simulink model "something_dumber"  (R2026b)
settings: Solver=ode23t  StopTime=simulation.timeSim  MaxStep=1/(5*solarPlant.converterSwitchingFrequency)  AbsTol=1e-3
PreLoadFcn:
  | run('something_dumb.mlx');
values from neighbouring files (symbols this model uses):
  P170_Imp = im(ix)    [P170_PV_Initialize.m]
  P170_Vmp = vm(ix)    [P170_PV_Initialize.m]
undefined symbols (not defined in the file or in its folder): battery, bms, bmsController, connectedLoad, dcVoltage, lunarCase, maxSoC, maxVdc, minIrrad, minSoC, minVdc, olTime, P170_T, sensor, solarPlant
libraries: nesl_utility x12, fl_lib x11, simulink x7, ee_lib x3, batteryecm_lib x1, simulink_extras x1, eePwmGenerator x1
(part 1 of 2)
settings Model: Creator=The MathWorks, Inc.  LastModifiedBy=aj26g
settings SolverCC: AutoScaleAbsTol=off
settings DataIOCC: DSMLogging=off  ReturnWorkspaceOutputs=off  SaveOutput=off  SaveTime=off  SignalLoggingName=SolarPVDCWithBattery_logDB
settings OptimizationCC: ReuseModelBlockBuffer=off
settings DebuggingCC: SymbolicDimsDataTypeCodeGenerationDiagnostic=none  UnderSpecifiedDimensionMsg=warning
settings SFSimCC: CustomCodeUndefinedFunction=UseInterfaceOnly
settings RTWCC: DLArmComputeVersion=19.05
settings SimscapeCC: SimscapeLogName=simlog_SolarPVDCWithBattery  SimscapeLogSimulationStatistics=on  SimscapeLogType=all  SimscapeUseEnergyAccounting=off

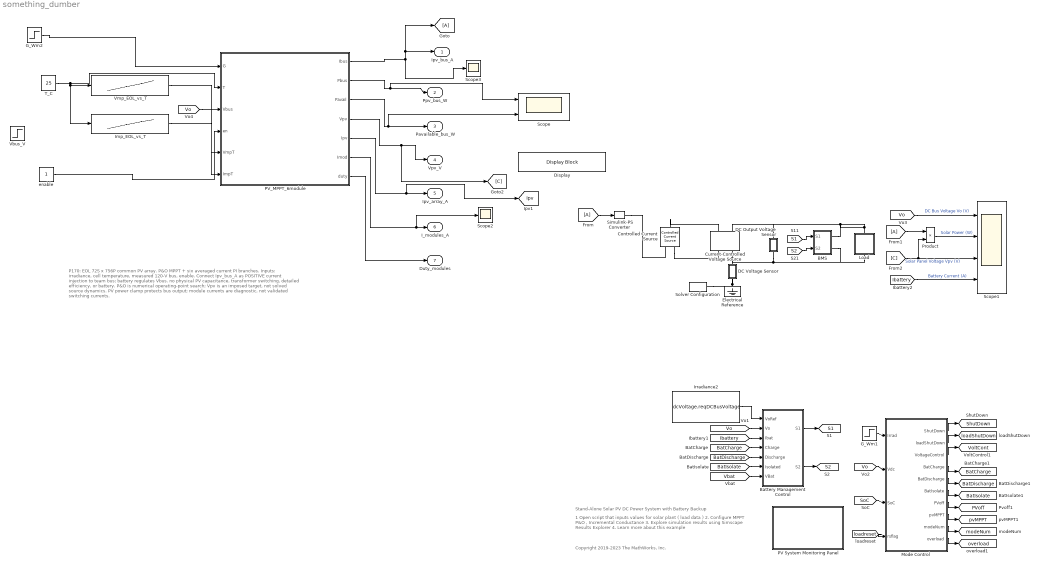
== system something_dumber ==
  note: 1 Open script that inputs values for solar plant ( load data )
      | 2. Configure MPPT P&O , Incremental Conductance
      | 3. Explore simulation results using Simscape Results Explorer
      | 4. Learn more about this example
  note: Stand-Alone Solar PV DC Power System with Battery Backup
  note: Copyright 2019-2023 The MathWorks, Inc.
  note: P170: EOL 72S x 756P common PV array. P&O MPPT + six averaged current PI branches.
      | Inputs: irradiance, cell temperature, measured 120-V bus, enable.
      | Connect Ipv_bus_A as POSITIVE current injection to team bus; battery regulates Vbus.
      |
      | no physical PV capacitance, transformer switching, detailed efficiency, or battery.
      | P&O is numerical operating-point search; Vpv is an imposed target, not solved source dynamics.
      | PV power clamp protects bus output; module currents are diagnostic, not validated switching currents.
  BMS : Subsystem
  Battery Management Control : Subsystem
  Controlled Current Source : fl_lib/Electrical/Electrical Sources/Controlled Current Source
  Current-Controlled Voltage Source : fl_lib/Electrical/Electrical Sources/Current-Controlled Voltage Source  K=1 Ohm  i1_specify=off  i1_priority=None  i1=0 A  i1_nominal_specify=off  i1_nominal_value=1  i1_nominal_unit=A  v2_specify=off  v2_priority=None  v2=0 V  v2_nominal_specify=off  v2_nominal_value=1  v2_nominal_unit=V
  DC Output Voltage Sensor : Subsystem
      mask Display: disp('v')
  DC Voltage Sensor : Subsystem
      mask Display: disp('v');
  Display : DisplayBlock  LabelPosition=Hide  Transparency=1  GridColor=[0.502, 0.502, 0.502]
  Electrical Reference : fl_lib/Electrical/Electrical Elements/Electrical Reference
  From : From
  From1 : From
  G_Wm1 : Step  Time=0.8  InitialValue=1367  FinalValue=700  SampleTime=0
  G_Wm2 : Step  Time=0.8  InitialValue=1367  FinalValue=700  SampleTime=0
  Goto : Goto
  Imp_EOL_vs_T : Lookup_n-D  NumberOfTableDimensions=1  BreakpointsForDimension1=P170_T  Table=P170_Imp  InternalRulePriority=Speed  RndMeth=Simplest
  Irradiance2 : Constant  Value=dcVoltage.reqDCBusVoltage
  Load : Subsystem
  Mode Control : Stateflow chart  TreatAsAtomicUnit=on
  PV System Monitoring Panel : Subsystem
  PV_MPPT_6module : MATLAB Function  TreatAsAtomicUnit=on
  Product : Product
  Scope : Scope  NumInputPorts=2
      settings: ActiveDisplayYMinimum=-1.4996053799360058  ActiveDisplayYMaximum=1.4239551585454688
  Scope1 : Scope  NumInputPorts=4
      settings: TimeSpan=simulation.timeSim  ActiveDisplayYMinimum=-72.27632  ActiveDisplayYMaximum=650.48692
  Scope2 : Scope
      settings: ActiveDisplayYMinimum=25.569170414602688  ActiveDisplayYMaximum=92.411823172385326  DataLoggingVariableName=ScopeData3
  Scope3 : Scope
      settings: ActiveDisplayYMinimum=153.59084488936233  ActiveDisplayYMaximum=552.88853741859577  DataLoggingVariableName=ScopeData2
  Simulink-PS Converter : nesl_utility/Simulink-PS Converter  PhysicalDomain=network_engine_domain  SubClassName=ps_input  LeftPortType=input  RightPortType=output  PseudoPeriodic=off  Frequencies=[]  NoiseDistribution=none  NoiseParameters=[]  Unit=1  AffineConversion=off  FilteringAndDerivatives=provide  SimscapeFilterOrder=1  InputFilterTimeConstant=0.001  UdotUserProvided=0
  Solver Configuration : nesl_utility/Solver Configuration  PhysicalDomain=network_engine_domain  SubClassName=solver  LeftPortType=input  RightPortType=generic  Tones=[]  Harmonics=[]  SimulateNoise=off  Profile=off  UseLocalSampling=off  EnableSwitchedLinearOptims=on  FrequencyDomain=off  UseCCode=off  RelTol=0.001  AbsTol=1e-06  MinStep=1e-09  ToWorkspace=off  RevertToSquareIcSolve=off  NumHomotopyIterations=100  PhasorMode=off  PhasorModeNumHarmonics=1  ConsistencySolver=NEWTON_FTOL  CanonicalOrdering=UNORDERED  OptimizeIntermediates=UNOPTIMIZED  MulticoreSolverChoice=BACKWARD_EULER  IndexReductionMethod=DerivativeReplacement  DoDC=off  ResidualTolerance=1e-9  ConsistencyTolSource=GLOBAL  ConsistencyAbsTol=0.001  ConsistencyRelTol=0.001  ConsistencyTolFactor=0.001  UseLocalSolver=off  LocalSolverChoice=NE_TRAPEZOIDAL_ADVANCER  ResolveIndetEquations=on  FunctionEvalNumThread=1  LocalSolverSampleTime=2e-6  DoFixedCost=off  MaxNonlinIter=10  MaxModeIter=2  ComputeImpulses=off  ImpulseIterations=2  LinearAlgebra=auto  LinearAlgebraNumThread=0  EquationFormulation=NE_TIME_EF  DelaysMemoryBudget=1024  AutomaticFiltering=on  FilteringTimeConstant=0.001  PartitionStorageMethod=AS_NEEDED  PartitionMemoryBudget=1024  PartitionMethod=FAST  MultibodyUseLocalSolver=off  MultibodyLocalSolverChoice=ODE1  MultibodyLocalSolverSampleTime=0.001
  T_C : Constant  Value=25
  Vbus_V : Step  Time=1.2  InitialValue=120  FinalValue=115  SampleTime=0
  Vmp_EOL_vs_T : Lookup_n-D  NumberOfTableDimensions=1  BreakpointsForDimension1=P170_T  Table=P170_Vmp  InternalRulePriority=Speed  RndMeth=Simplest
  enable : Constant
  Ipv_bus_A : Outport
  Ppv_bus_W : Outport  Port=2
  Pavailable_bus_W : Outport  Port=3
  Vpv_V : Outport  Port=4
  Ipv_array_A : Outport  Port=5
  I_modules_A : Outport  Port=6
  Duty_modules : Outport  Port=7
  tag scope: BatCharge=global, BatDischarge=global, BatIsolate=global, Ipv=global, PVoff=global, S1=global, S2=global, ShutDown=global, VoltCont=global, loadShutDown=global, modeNum=global, overload=global, pvMPPT=global
  wires:
  Mode Control/5(BatDischarge) -> [BatDischarge]
  [C] -> Scope1/3, Product/2  "Solar Panel Voltage Vpv (V)"
  Battery Management Control/2(S2) -> [S2]
  [Ibattery] -> Battery Management Control/3(Ibat)
  Product/1 -> Scope1/2  "Solar Power (W)"
  [Vbat] -> Battery Management Control/7(VBat)
  Mode Control/2(loadShutDown) -> [loadShutDown]
  Mode Control/9(modeNum) -> [modeNum]
  [BatDischarge] -> Battery Management Control/5(Discharge)
  Mode Control/10(overload) -> [overload]
  From1/1 -> Product/1
  Mode Control/1(ShutDown) -> [ShutDown]
  Mode Control/3(VoltageControl) -> [VoltCont]
  [BatIsolate] -> Battery Management Control/6(Isolated)
  [Vo] -> Mode Control/2(Vdc)
  Mode Control/8(pvMPPT) -> [pvMPPT]
  [loadreset] -> Mode Control/4(rsflag)
  [SoC] -> Mode Control/3(SoC)
  Mode Control/6(BatIsolate) -> [BatIsolate]
  Irradiance2/1 -> Battery Management Control/1(VoRef)
  G_Wm1/1 -> Mode Control/1(Irrad)
  Mode Control/7(PVoff) -> [PVoff]
  [Vo] -> Scope1/1  "DC Bus Voltage Vo (V)"
  Mode Control/4(BatCharge) -> [BatCharge]
  Battery Management Control/1(S1) -> [S1]
  [Ibattery] -> Scope1/4  "Battery Current (A)"
  [Vo] -> Battery Management Control/2(Vo)
  [S2] -> BMS/2(S2)
  [BatCharge] -> Battery Management Control/4(Charge)
  [S1] -> BMS/1(S1)
  PV_MPPT_6module/6(Imod) -> Scope2/1, I_modules_A/1
  PV_MPPT_6module/1(Ibus) -> Scope3/1, Goto/1, Ipv_bus_A/1
  G_Wm2/1 -> PV_MPPT_6module/1(G)
  PV_MPPT_6module/4(Vpv) -> [C], Vpv_V/1
  PV_MPPT_6module/5(Ipv) -> [Ipv], Ipv_array_A/1
  PV_MPPT_6module/7(duty) -> Duty_modules/1
  Imp_EOL_vs_T/1 -> PV_MPPT_6module/6(ImpT)
  PV_MPPT_6module/3(Pavail) -> Scope/2, Pavailable_bus_W/1
  enable/1 -> PV_MPPT_6module/4(en)
  PV_MPPT_6module/2(Pbus) -> Scope/1, Ppv_bus_W/1
  T_C/1 -> Vmp_EOL_vs_T/1, Imp_EOL_vs_T/1, PV_MPPT_6module/2(T)
  Vmp_EOL_vs_T/1 -> PV_MPPT_6module/5(VmpT)
  From/1 -> Simulink-PS Converter/1
  [Vo] -> PV_MPPT_6module/3(Vbus)
  connections:
  Load/LConn1 -- DC Output Voltage Sensor/RConn1 -- Current-Controlled Voltage Source/LConn2 -- BMS/RConn1
  Solver Configuration/RConn1 -- Electrical Reference/LConn1 -- DC Voltage Sensor/LConn1
  BMS/RConn2 -- Load/RConn1 -- Current-Controlled Voltage Source/RConn2 -- DC Voltage Sensor/RConn1 -- DC Output Voltage Sensor/LConn1
  Simulink-PS Converter/RConn1 -- Controlled Current Source/RConn1
  Controlled Current Source/LConn1 -- Current-Controlled Voltage Source/LConn1
  Controlled Current Source/RConn2 -- Current-Controlled Voltage Source/RConn1

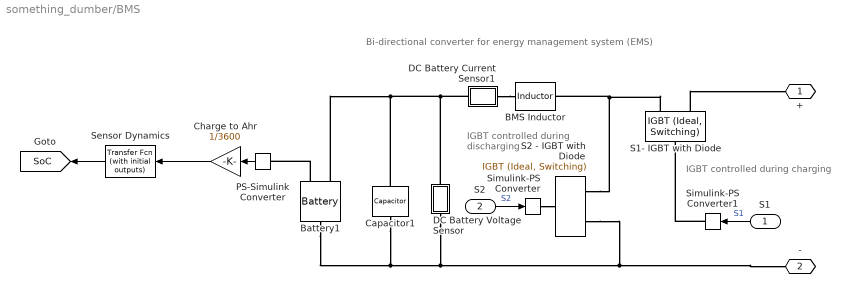
== system something_dumber/BMS ==
  note: IGBT controlled during charging
  note: Bi-directional converter for energy management system (EMS)
  note: IGBT controlled during discharging
  S1 : Inport
  S2 : Inport  Port=2
  BMS Inductor : fl_lib/Electrical/Electrical Elements/Inductor  l=bms.batteryChargingInductor H  r=bms.batteryChargingInductorResistance Ohm  g=1e-9 1/Ohm  i_specify=off  i_priority=High  i=0 A  i_nominal_specify=off  i_nominal_value=1  i_nominal_unit=A  v_specify=off  v_priority=High  v=0 V  v_nominal_specify=off  v_nominal_value=1  v_nominal_unit=V  i_L_specify=on  i_L_priority=High  i_L=0 A  i_L_nominal_specify=off  i_L_nominal_value=1  i_L_nominal_unit=A
      settings: LogSimulationData=on
  Battery1 : batteryecm_lib/Battery  Vnom=battery.nominalBatteryVoltage V  prm_dir=1  R1_dis=2 Ohm  R1_ch=2 Ohm  R1=0.01 Ohm  prm_AH=2  AH=connectedLoad.batteryAmpHr hr*A  V1=battery.minBatteryNominalVoltage V  AH1=connectedLoad.batteryAmpHr*0.2 hr*A  prm_R2=2  R2=2000 Ohm  Tmeas=298.15 K  charge_measurement_port=simscape.enum.battery.enable.yes  prm_dyn=1  Rp1=0.005 Ohm  tau1=30 s  Rp2=0.005 Ohm  tau2=30 s  Rp3=0.005 Ohm  tau3=30 s  Rp4=0.005 Ohm  tau4=30 s  Rp5=0.005 Ohm  tau5=30 s  prm_fade=1  N_fade=100  AH_fade=45 hr*A  R1_fade=2.02 Ohm  R1_ch_fade=2.02 Ohm  V1_fade=10.35 V  prm_age=1  prm_age_OCV=1  OCV_age=0.9  SOC_age=60  Tmeas_age=298.15 K  delta_time_age_vec=[0] d  temperature_age_vec=[273] K  OCV_scaling_age=2.2134e6  OCV_offset_age=1.632e6  temp_exp_age=0.515833569 V  t_exp_age=0.75  Vnom_T2=12 V  R1_T2=2.2 Ohm  R1_T2_dis=2.2 Ohm  R1_T2_ch=2.2 Ohm  V1_T2=11.4 V  R2_T2=2200 Ohm  Rp1_T2=0.005 Ohm  tau1_T2=30 s  Rp2_T2=0.005 Ohm  tau2_T2=30 s  Rp3_T2=0.005 Ohm  tau3_T2=30 s  Rp4_T2=0.005 Ohm  tau4_T2=30 s  Rp5_T2=0.005 Ohm  tau5_T2=30 s  Tmeas2=273.15 K  thermal_port=simscape.enum.thermaleffects.omit  thermal_mass=30000 J/K  i_specify=off  i_priority=None  i=0 A  i_nominal_specify=off  i_nominal_value=1  i_nominal_unit=A  v_specify=off  v_priority=None  v=0 V  v_nominal_specify=off  v_nominal_value=1  v_nominal_unit=V  charge_specify=on  charge_priority=High  charge=batteryInitialStateOfCharge hr*A  charge_nominal_specify=off  charge_nominal_value=1  charge_nominal_unit=A*hr  num_cycles_specify=off  num_cycles_priority=High  num_cycles=0  num_cycles_nominal_specify=off  num_cycles_nominal_value=1  num_cycles_nominal_unit=1  temperature_specify=off  temperature_priority=High  temperature=298.15 K  temperature_nominal_specify=off  temperature_nominal_value=1  temperature_nominal_unit=K
  Capacitor1 : fl_lib/Electrical/Electrical Elements/Capacitor  c=boost.outputCapacitor F  r=1e-6 Ohm  g=0 1/Ohm  i_specify=off  i_priority=None  i=0 A  i_nominal_specify=off  i_nominal_value=1  i_nominal_unit=A  v_specify=off  v_priority=None  v=0 V  v_nominal_specify=off  v_nominal_value=1  v_nominal_unit=V  vc_specify=on  vc_priority=High  vc=batteryInputCapacitorInitialVoltage V  vc_nominal_specify=off  vc_nominal_value=1  vc_nominal_unit=V
  Charge to Ahr : Gain  Gain=1/3600
  DC Battery Current Sensor1 : Subsystem
      mask Display: disp('i');
  DC Battery Voltage Sensor : Subsystem
      mask Display: disp('v');
  PS-Simulink Converter : nesl_utility/PS-Simulink Converter  PhysicalDomain=network_engine_domain  SubClassName=ps_output  LeftPortType=input  RightPortType=output  PseudoPeriodic=off  Frequencies=[]  VectorFormat=1-D array  Unit=inherit  AffineConversion=off
  S1- IGBT with Diode : ee_lib/Semiconductors & Converters/IGBT (Ideal, Switching)  port_option=ee.enum.controlport.ps  Vf=0.1 V  Ron=0.001 Ohm  Goff=1e-5 1/Ohm  Vth=2.5 V  diode_param=2  diode_Vf=0.1 V  diode_Ron=0.001 Ohm  diode_Goff=1e-5 1/Ohm  diode_C=50e-9 F  diode_iRM=-235 A  diode_iF=300 A  diode_idot=-50 A/us  diode_trr_param=1  diode_trr_factor=3  diode_trr=15 us  diode_Qrr=1500 s*uA  ice_specify=off  ice_priority=None  ice=0 A  ice_nominal_specify=off  ice_nominal_value=1  ice_nominal_unit=A  vce_specify=off  vce_priority=None  vce=0 V  vce_nominal_specify=off  vce_nominal_value=1  vce_nominal_unit=V  vge_specify=off  vge_priority=None  vge=0 V  vge_nominal_specify=off  vge_nominal_value=1  vge_nominal_unit=V  thermal_loss_option=ee.enum.converters.thermalLossOption.constantvalues  Von_data=[0, .1, .6, .8, 1, 1.3, 1.6, 2, 2.4; 0, .1, .7, 1, 1.2, 1.5, 1.9, 2.4, 2.8] V  Tj=[298.15, 398.15] K  Iout_data=[0, .1, 1, 5, 10, 20, 40, 70, 100] A  tabulateWithVce=false  Eon_data=[0, .0024, .024, .12, .2, .48, 1.04, 2.16, 3.24; 0, .003, .03, .15, .25, .6, 1.3, 2.7, 4.05] * 1e-3 J  Eoff_data=[0, .0007, .0066, .033, .066, .17, .33, .83, 1.5; 0, .001, .01, .05, .1, .25, .5, 1.2, 2.2] * 1e-3 J  Eon_data_3D=[zeros(2, 9, 3)] J  Eoff_data_3D=[zeros(2, 9, 3)] J  Tj_loss=[298.15, 398.15] K  Iout_data_loss=[0, .1, 1, 5, 10, 20, 40, 70, 100] A  Vce_loss=[0, 150, 300] V  Eon_scalar=22.86e-3 J  Eoff_scalar=17.14e-3 J  Voff=300 V  Iout_scalar=600 A  useCurrentFromPreviousCycle=true  currentMeasDelay=0 s  useVoltageFromPreviousCycle=true  voltageMeasDelay=0 s  diodeModelType=ee.enum.converters.diodeModelType.pwl  diodeTableType=ee.enum.diode.tableType.IfMat  diode_ReverseIVType=ee.enum.diode.diodeReverseIV.constant  diode_IfMat=[.07, .12, .19, 1.75, 4.24, 7.32, 11.2; .16, .3, .72, 2.14, 4.02, 6.35, 9.12] A  diode_VfMat=[.9, 1.15, 1.25, 1.5, 1.75, 2.17, 2.6, 2.85; .58, .68, .75, 1.1, 1.38, 1.77, 2.27, 2.7] V  diode_TjVec=[25, 125] degC  diode_VfVec=[.5, .7, .9, 1.3, 1.7, 2.1, 2.5] V  diode_IfVec=[.1, .2, .5, 1, 2, 4, 7, 10] A  diode_IrMat=[1e-06, 2e-06, 5e-06, 1e-05, 2.5e-05, 5e-05, .0001; 2e-06, 5e-06, 1e-05, 4e-05, 8e-05, .0002, .0005] A  diode_VrMat=[10, 100, 200, 250, 300, 325, 350; 10, 70, 160, 220, 270, 300, 320] V  diode_VrVec=[10, 20, 40, 50, 70, 80, 100] V  diode_IrVec=[1e-06, 2e-06, 5e-06, 1e-05, 2e-05, 5e-05, .0001] A  diode_Vr=-600 V  diode_Ls=150 nH  diode_Erec=0.03 J  diode_rec_loss_model=ee.enum.diode.reverseRecoveryModelTabulateUpTo3D.fixed  diode_ErecVal=0 J  diode_scaleWithIandV=true  diode_ErecMat=zeros(2, 3) J  diodeErecMat3D=zeros(2, 3, 2) J  diode_TjrecVec=[298.15, 398.15] K  diode_IfrecVec=[.1, 1, 10] A  diodeVrecVec=[0, 100] V  diode_IrecVal=10 A  diode_VrecVal=10 V  diode_tFilter=1 / 1000 / 100 s  separateThermalPortForDiode=false  thermal_network_parameterization=ee.enum.thermalNetworkTopology.external  Rth=[.08, .5] K/W  Rth_Cauer=[.08, .1, .5] K/W  Rth_Foster=[.08, .14, .22, .16] K/W  thermal_mass_parameterization=ee.enum.thermalNetwork.timeconstant  thermal_mass=[.01, .5] J/K  thermal_mass_Cauer=[.01, .1, .5] J/K  thermal_mass_Foster=[.001, .005, .05, .5] J/K  thermal_time_constant=[.001, .2] s  thermal_time_constant_Cauer=[.001, .1, .2] s  thermal_time_constant_Foster=[7e-05, .0007, .01, .08] s  thermal_mass_initial_temperatures=[25, 25] degC  thermal_mass_initial_temperatures_Cauer=[25, 25, 25] degC  junction_thermal_mass=0.01 J/K  Tvec_initial_Foster=[25, 25, 25, 25] degC  RthDiode=[.03, .2] K/W  RthCauerDiode=[.03, .1, .2] K/W  RthFosterDiode=[.03, .2] K/W  thermalMassDiode=[3, 25] J/K  thermalMassCauerDiode=[3, 10, 25] J/K  thermalMassFosterDiode=[33, 50] J/K  thermalTauDiode=[.1, 5] s  thermalTauCauerDiode=[.1, 1, 5] s  thermalTauFosterDiode=[1, 10] s  thermalMassInitTempDiode=[25, 25] degC  thermalMassInitTempCauerDiode=[25, 25, 25] degC  junctionthermalMassDiode=0.1 J/K  TVecInitialFosterDiode=[25, 25] degC  no_thermal_network=0  IGBT_junction_temperature_specify=off  IGBT_junction_temperature_priority=None  IGBT_junction_temperature=25 degC  IGBT_junction_temperature_nominal_specify=off  IGBT_junction_temperature_nominal_value=1  IGBT_junction_temperature_nominal_unit=degC  diode_junction_temperature_specify=off  diode_junction_temperature_priority=None  diode_junction_temperature=25 degC  diode_junction_temperature_nominal_specify=off  diode_junction_temperature_nominal_value=1  diode_junction_temperature_nominal_unit=degC  Qj_specify=off  Qj_priority=None  Qj=0 W  Qj_nominal_specify=off  Qj_nominal_value=1  Qj_nominal_unit=W  accumulatedSwitchingLosses_specify=off  accumulatedSwitchingLosses_priority=None  accumulatedSwitchingLosses=0 J
  S2 - IGBT with Diode : ee_lib/Semiconductors & Converters/IGBT (Ideal, Switching)  port_option=ee.enum.controlport.ps  Vf=0.1 V  Ron=0.001 Ohm  Goff=1e-5 1/Ohm  Vth=2.5 V  diode_param=2  diode_Vf=0.1 V  diode_Ron=0.001 Ohm  diode_Goff=1e-5 1/Ohm  diode_C=50e-9 F  diode_iRM=-235 A  diode_iF=300 A  diode_idot=-50 A/us  diode_trr_param=1  diode_trr_factor=3  diode_trr=15 us  diode_Qrr=1500 s*uA  ice_specify=off  ice_priority=None  ice=0 A  ice_nominal_specify=off  ice_nominal_value=1  ice_nominal_unit=A  vce_specify=off  vce_priority=None  vce=0 V  vce_nominal_specify=off  vce_nominal_value=1  vce_nominal_unit=V  vge_specify=off  vge_priority=None  vge=0 V  vge_nominal_specify=off  vge_nominal_value=1  vge_nominal_unit=V  thermal_loss_option=ee.enum.converters.thermalLossOption.constantvalues  Von_data=[0, .1, .6, .8, 1, 1.3, 1.6, 2, 2.4; 0, .1, .7, 1, 1.2, 1.5, 1.9, 2.4, 2.8] V  Tj=[298.15, 398.15] K  Iout_data=[0, .1, 1, 5, 10, 20, 40, 70, 100] A  tabulateWithVce=false  Eon_data=[0, .0024, .024, .12, .2, .48, 1.04, 2.16, 3.24; 0, .003, .03, .15, .25, .6, 1.3, 2.7, 4.05] * 1e-3 J  Eoff_data=[0, .0007, .0066, .033, .066, .17, .33, .83, 1.5; 0, .001, .01, .05, .1, .25, .5, 1.2, 2.2] * 1e-3 J  Eon_data_3D=[zeros(2, 9, 3)] J  Eoff_data_3D=[zeros(2, 9, 3)] J  Tj_loss=[298.15, 398.15] K  Iout_data_loss=[0, .1, 1, 5, 10, 20, 40, 70, 100] A  Vce_loss=[0, 150, 300] V  Eon_scalar=22.86e-3 J  Eoff_scalar=17.14e-3 J  Voff=300 V  Iout_scalar=600 A  useCurrentFromPreviousCycle=true  currentMeasDelay=0 s  useVoltageFromPreviousCycle=true  voltageMeasDelay=0 s  diodeModelType=ee.enum.converters.diodeModelType.pwl  diodeTableType=ee.enum.diode.tableType.IfMat  diode_ReverseIVType=ee.enum.diode.diodeReverseIV.constant  diode_IfMat=[.07, .12, .19, 1.75, 4.24, 7.32, 11.2; .16, .3, .72, 2.14, 4.02, 6.35, 9.12] A  diode_VfMat=[.9, 1.15, 1.25, 1.5, 1.75, 2.17, 2.6, 2.85; .58, .68, .75, 1.1, 1.38, 1.77, 2.27, 2.7] V  diode_TjVec=[25, 125] degC  diode_VfVec=[.5, .7, .9, 1.3, 1.7, 2.1, 2.5] V  diode_IfVec=[.1, .2, .5, 1, 2, 4, 7, 10] A  diode_IrMat=[1e-06, 2e-06, 5e-06, 1e-05, 2.5e-05, 5e-05, .0001; 2e-06, 5e-06, 1e-05, 4e-05, 8e-05, .0002, .0005] A  diode_VrMat=[10, 100, 200, 250, 300, 325, 350; 10, 70, 160, 220, 270, 300, 320] V  diode_VrVec=[10, 20, 40, 50, 70, 80, 100] V  diode_IrVec=[1e-06, 2e-06, 5e-06, 1e-05, 2e-05, 5e-05, .0001] A  diode_Vr=-600 V  diode_Ls=150 nH  diode_Erec=0.03 J  diode_rec_loss_model=ee.enum.diode.reverseRecoveryModelTabulateUpTo3D.fixed  diode_ErecVal=0 J  diode_scaleWithIandV=true  diode_ErecMat=zeros(2, 3) J  diodeErecMat3D=zeros(2, 3, 2) J  diode_TjrecVec=[298.15, 398.15] K  diode_IfrecVec=[.1, 1, 10] A  diodeVrecVec=[0, 100] V  diode_IrecVal=10 A  diode_VrecVal=10 V  diode_tFilter=1 / 1000 / 100 s  separateThermalPortForDiode=false  thermal_network_parameterization=ee.enum.thermalNetworkTopology.external  Rth=[.08, .5] K/W  Rth_Cauer=[.08, .1, .5] K/W  Rth_Foster=[.08, .14, .22, .16] K/W  thermal_mass_parameterization=ee.enum.thermalNetwork.timeconstant  thermal_mass=[.01, .5] J/K  thermal_mass_Cauer=[.01, .1, .5] J/K  thermal_mass_Foster=[.001, .005, .05, .5] J/K  thermal_time_constant=[.001, .2] s  thermal_time_constant_Cauer=[.001, .1, .2] s  thermal_time_constant_Foster=[7e-05, .0007, .01, .08] s  thermal_mass_initial_temperatures=[25, 25] degC  thermal_mass_initial_temperatures_Cauer=[25, 25, 25] degC  junction_thermal_mass=0.01 J/K  Tvec_initial_Foster=[25, 25, 25, 25] degC  RthDiode=[.03, .2] K/W  RthCauerDiode=[.03, .1, .2] K/W  RthFosterDiode=[.03, .2] K/W  thermalMassDiode=[3, 25] J/K  thermalMassCauerDiode=[3, 10, 25] J/K  thermalMassFosterDiode=[33, 50] J/K  thermalTauDiode=[.1, 5] s  thermalTauCauerDiode=[.1, 1, 5] s  thermalTauFosterDiode=[1, 10] s  thermalMassInitTempDiode=[25, 25] degC  thermalMassInitTempCauerDiode=[25, 25, 25] degC  junctionthermalMassDiode=0.1 J/K  TVecInitialFosterDiode=[25, 25] degC  no_thermal_network=0  IGBT_junction_temperature_specify=off  IGBT_junction_temperature_priority=None  IGBT_junction_temperature=25 degC  IGBT_junction_temperature_nominal_specify=off  IGBT_junction_temperature_nominal_value=1  IGBT_junction_temperature_nominal_unit=degC  diode_junction_temperature_specify=off  diode_junction_temperature_priority=None  diode_junction_temperature=25 degC  diode_junction_temperature_nominal_specify=off  diode_junction_temperature_nominal_value=1  diode_junction_temperature_nominal_unit=degC  Qj_specify=off  Qj_priority=None  Qj=0 W  Qj_nominal_specify=off  Qj_nominal_value=1  Qj_nominal_unit=W  accumulatedSwitchingLosses_specify=off  accumulatedSwitchingLosses_priority=None  accumulatedSwitchingLosses=0 J
  Sensor Dynamics : simulink_extras/Additional Linear/Transfer Fcn (with initial outputs)  N=[1]  D=[1/sensor.samplingFreq 1]  Y0=minSoC  U0=0
  Simulink-PS Converter : nesl_utility/Simulink-PS Converter  PhysicalDomain=network_engine_domain  SubClassName=ps_input  LeftPortType=input  RightPortType=output  PseudoPeriodic=off  Frequencies=[]  NoiseDistribution=none  NoiseParameters=[]  Unit=1  AffineConversion=off  FilteringAndDerivatives=provide  SimscapeFilterOrder=1  InputFilterTimeConstant=0.001  UdotUserProvided=0
  Simulink-PS Converter1 : nesl_utility/Simulink-PS Converter  PhysicalDomain=network_engine_domain  SubClassName=ps_input  LeftPortType=input  RightPortType=output  PseudoPeriodic=off  Frequencies=[]  NoiseDistribution=none  NoiseParameters=[]  Unit=1  AffineConversion=off  FilteringAndDerivatives=provide  SimscapeFilterOrder=1  InputFilterTimeConstant=0.001  UdotUserProvided=0
  + : PMIOPort  Side=Right
  - : PMIOPort  Port=2  Side=Right
  tag scope: SoC=global
  wires:
  S2/1 -> Simulink-PS Converter/1  "S2"
  S1/1 -> Simulink-PS Converter1/1  "S1"
  PS-Simulink Converter/1 -> Charge to Ahr/1
  Sensor Dynamics/1 -> [SoC]
  Charge to Ahr/1 -> Sensor Dynamics/1
  connections:
  S2 - IGBT with Diode/RConn2 -- Battery1/RConn1 -- Capacitor1/RConn1 -- DC Battery Voltage Sensor/LConn1 -- -/RConn1
  S2 - IGBT with Diode/RConn1 -- S1- IGBT with Diode/RConn2 -- BMS Inductor/RConn1
  S1- IGBT with Diode/RConn1 -- +/RConn1
  Simulink-PS Converter/RConn1 -- S2 - IGBT with Diode/LConn1
  Battery1/LConn2 -- PS-Simulink Converter/LConn1
  Simulink-PS Converter1/RConn1 -- S1- IGBT with Diode/LConn1
  DC Battery Current Sensor1/RConn1 -- BMS Inductor/LConn1
  DC Battery Current Sensor1/LConn1 -- DC Battery Voltage Sensor/RConn1 -- Battery1/LConn1 -- Capacitor1/LConn1

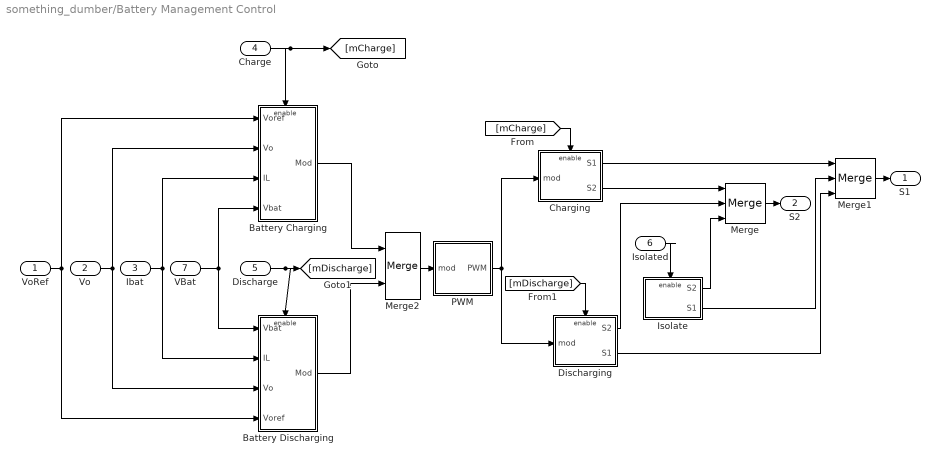
== system something_dumber/Battery Management Control ==
  VoRef : Inport
  Vo : Inport  Port=2
  Ibat : Inport  Port=3
  Charge : Inport  Port=4
  Discharge : Inport  Port=5
  Isolated : Inport  Port=6
  VBat : Inport  Port=7
  Battery Charging : Subsystem
  Battery Discharging : Subsystem
  Charging : Subsystem  TreatAsAtomicUnit=on
  Discharging : Subsystem  TreatAsAtomicUnit=on
  Isolate : Subsystem  TreatAsAtomicUnit=on
  Merge : Merge  Inputs=3
  Merge1 : Merge  Inputs=3
  Merge2 : Merge
  PWM : Subsystem
  S1 : Outport
  S2 : Outport  Port=2
  wires:
  Charging/2(S2) -> Merge/1
  Discharging/1(S2) -> Merge/2
  Charging/1(S1) -> Merge1/1
  Isolate/1(S2) -> Merge/3
  Isolate/2(S1) -> Merge1/2
  Discharging/2(S1) -> Merge1/3
  Merge1/1 -> S1/1
  Isolated/1 -> Isolate/Enable
  Vo/1 -> Battery Charging/2(Vo), Battery Discharging/3(Vo)
  Ibat/1 -> Battery Charging/3(IL), Battery Discharging/2(IL)
  Battery Charging/1(Mod) -> Merge2/1
  Battery Discharging/1(Mod) -> Merge2/2
  Merge/1 -> S2/1
  Charge/1 -> [mCharge], Battery Charging/Enable
  Discharge/1 -> Battery Discharging/Enable, [mDischarge]
  [mCharge] -> Charging/Enable
  [mDischarge] -> Discharging/Enable
  PWM/1(PWM) -> Charging/1(mod), Discharging/1(mod)
  Merge2/1 -> PWM/1(mod)
  VoRef/1 -> Battery Charging/1(Voref), Battery Discharging/4(Voref)
  VBat/1 -> Battery Discharging/1(Vbat), Battery Charging/4(Vbat)

== system something_dumber/DC Output Voltage Sensor ==
  PS-Simulink Converter : nesl_utility/PS-Simulink Converter  PhysicalDomain=network_engine_domain  SubClassName=ps_output  LeftPortType=input  RightPortType=output  PseudoPeriodic=off  Frequencies=[]  VectorFormat=1-D array  Unit=1  AffineConversion=off
  Sensor dynamics : TransferFcn  Numerator=1  Denominator=[1/sensor.samplingFreq 1]
  Voltage Sensor : fl_lib/Electrical/Electrical Sensors/Voltage Sensor
  - : PMIOPort  Side=Left
  + : PMIOPort  Port=2  Side=Right
  tag scope: Vo=global
  wires:
  PS-Simulink Converter/1 -> Sensor dynamics/1
  Sensor dynamics/1 -> [Vo]
  connections:
  Voltage Sensor/RConn2 -- -/RConn1
  Voltage Sensor/RConn1 -- PS-Simulink Converter/LConn1
  Voltage Sensor/LConn1 -- +/RConn1

== system something_dumber/DC Voltage Sensor ==
  PS-Simulink Converter : nesl_utility/PS-Simulink Converter  PhysicalDomain=network_engine_domain  SubClassName=ps_output  LeftPortType=input  RightPortType=output  PseudoPeriodic=off  Frequencies=[]  VectorFormat=1-D array  Unit=1  AffineConversion=off
  Sensor dynamics : TransferFcn  Numerator=1  Denominator=[1/sensor.samplingFreq 1]
  Voltage Sensor : fl_lib/Electrical/Electrical Sensors/Voltage Sensor
      settings: LogSimulationData=on
  - : PMIOPort  Side=Left
  + : PMIOPort  Port=2  Side=Right
  tag scope: Vpv=global
  wires:
  PS-Simulink Converter/1 -> Sensor dynamics/1
  Sensor dynamics/1 -> [Vpv]
  connections:
  Voltage Sensor/LConn1 -- +/RConn1
  Voltage Sensor/RConn1 -- PS-Simulink Converter/LConn1
  Voltage Sensor/RConn2 -- -/RConn1

== system something_dumber/Load ==
  AC Current Sensor2 : Subsystem
      mask Display: disp('i');
  Load : Subsystem
  Load Flag : Subsystem
  Load Resistance : fl_lib/Electrical/Electrical Elements/Variable Resistor  Rmin=0 Ohm  thermalEnable=false  thermal_mass=1 J/K  i_specify=off  i_priority=None  i=5 A  i_nominal_specify=off  i_nominal_value=1  i_nominal_unit=A  v_specify=off  v_priority=None  v=0 V  v_nominal_specify=off  v_nominal_value=1  v_nominal_unit=V  T_specify=off  T_priority=None  T=300 K  T_nominal_specify=off  T_nominal_value=1  T_nominal_unit=K
  SPST Switch : ee_lib/Switches & Breakers/SPST Switch  R_closed=0.01 Ohm  G_open=1e-6 S  Threshold=0.5 V  Width=0 V  model_dynamics=0  t_on=1e-3 s  t_off=1e-3 s  initial_vT=0 V
  + : PMIOPort  Side=Left
  - : PMIOPort  Port=2  Side=Right
  connections:
  +/RConn1 -- SPST Switch/LConn2
  Load Resistance/LConn2 -- AC Current Sensor2/LConn1
  Load Resistance/RConn1 -- -/RConn1
  Load/RConn1 -- Load Resistance/LConn1
  Load Flag/RConn1 -- SPST Switch/LConn1
  AC Current Sensor2/RConn1 -- SPST Switch/RConn1

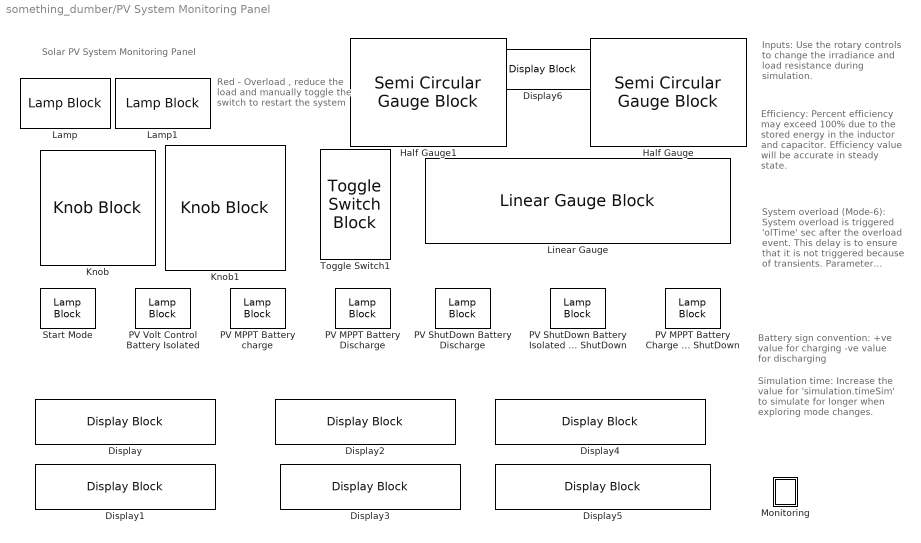
== system something_dumber/PV System Monitoring Panel ==
  note: Red - Overload , reduce the load and manually toggle the switch to restart the system
  note: Solar PV System Monitoring Panel
  note: Simulation time:
      | Increase the value for 'simulation.timeSim' to simulate for longer when exploring mode changes.
  note: Inputs:
      | Use the rotary controls to change the irradiance and load resistance during simulation.
  note: System overload (Mode-6):
      | System overload is triggered 'olTime' sec after the overload event. This delay is to ensure that it is not triggered because of transients. Parameter 'olTime' can be modified in the supporting livescript.
  note: Efficiency:
      | Percent efficiency may exceed 100% due to the stored energy in the inductor and capacitor. Efficiency value will be accurate in steady state.
  note: Battery sign convention:
      | +ve value for charging
      | -ve value for discharging
  Display{,1..6} (7 alike) : DisplayBlock  Transparency=1  GridColor=[0.502, 0.502, 0.502]
  Half Gauge : SemiCircularGaugeBlock  ScaleMin=20  FontColor=[0.0, 0.0, 0.0]
  Half Gauge1 : SemiCircularGaugeBlock  FontColor=[0.0, 0.0, 0.0]
  Knob : KnobBlock  ScaleMin=150  ScaleMax=1000
  Knob1 : KnobBlock  ScaleMin=0.15  ScaleMax=20
  Lamp : LampBlock  DefaultColor=[192.0, 192.0, 192.0]
  Lamp1 : LampBlock  DefaultColor=[192.0, 192.0, 192.0]
  Linear Gauge : LinearGaugeBlock  ScaleMin=-100  FontColor=[0.0, 0.0, 0.0]
  Monitoring : Subsystem
  PV MPPT Battery Charge Load ShutDown : LampBlock  DefaultColor=[192.0, 192.0, 192.0]
  PV MPPT Battery Discharge : LampBlock  DefaultColor=[192.0, 192.0, 192.0]
  PV MPPT Battery charge : LampBlock  DefaultColor=[192.0, 192.0, 192.0]
  PV ShutDown Battery Discharge : LampBlock  DefaultColor=[192.0, 192.0, 192.0]
  PV ShutDown Battery Isolated System ShutDown : LampBlock  DefaultColor=[192.0, 192.0, 192.0]
  PV Volt Control Battery Isolated : LampBlock  DefaultColor=[192.0, 192.0, 192.0]
  Start Mode : LampBlock  DefaultColor=[192.0, 192.0, 192.0]
  Toggle Switch1 : ToggleSwitchBlock

== system something_dumber/BMS/DC Battery Current Sensor1 ==
  Current Sensor : fl_lib/Electrical/Electrical Sensors/Current Sensor
  PS-Simulink Converter : nesl_utility/PS-Simulink Converter  PhysicalDomain=network_engine_domain  SubClassName=ps_output  LeftPortType=input  RightPortType=output  PseudoPeriodic=off  Frequencies=[]  VectorFormat=1-D array  Unit=1  AffineConversion=off
  Sensor dynamics : TransferFcn  Numerator=1  Denominator=[1/sensor.samplingFreq 1]
  - : PMIOPort  Side=Left
  + : PMIOPort  Port=2  Side=Right
  tag scope: Ibattery=global
  wires:
  PS-Simulink Converter/1 -> Sensor dynamics/1
  Sensor dynamics/1 -> [Ibattery]
  connections:
  Current Sensor/RConn1 -- PS-Simulink Converter/LConn1
  +/RConn1 -- Current Sensor/LConn1
  Current Sensor/RConn2 -- -/RConn1

== system something_dumber/BMS/DC Battery Voltage Sensor ==
  PS-Simulink Converter : nesl_utility/PS-Simulink Converter  PhysicalDomain=network_engine_domain  SubClassName=ps_output  LeftPortType=input  RightPortType=output  PseudoPeriodic=off  Frequencies=[]  VectorFormat=1-D array  Unit=1  AffineConversion=off
  Sensor dynamics : TransferFcn  Numerator=1  Denominator=[1/sensor.samplingFreq 1]
  Voltage Sensor : fl_lib/Electrical/Electrical Sensors/Voltage Sensor
      settings: LogSimulationData=on
  - : PMIOPort  Side=Left
  + : PMIOPort  Port=2  Side=Right
  tag scope: Vbat=global
  wires:
  PS-Simulink Converter/1 -> Sensor dynamics/1
  Sensor dynamics/1 -> [Vbat]
  connections:
  Voltage Sensor/LConn1 -- +/RConn1
  Voltage Sensor/RConn1 -- PS-Simulink Converter/LConn1
  Voltage Sensor/RConn2 -- -/RConn1

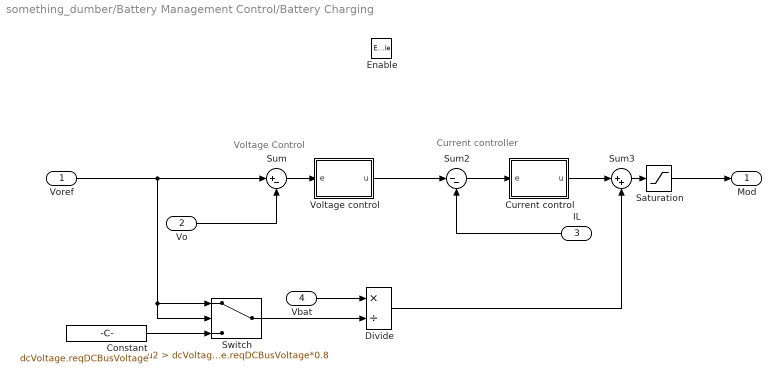
== system something_dumber/Battery Management Control/Battery Charging ==
  note: Current controller
  note: Voltage Control
  Voref : Inport
  Vo : Inport  Port=2
  IL : Inport  Port=3
  Vbat : Inport  Port=4
  Enable : EnablePort  StatesWhenEnabling=reset
  Constant : Constant  Value=dcVoltage.reqDCBusVoltage
  Current control : Subsystem
  Divide : Product  Inputs=*/
  Saturation : Saturate  UpperLimit=1  LowerLimit=0
  Sum : Sum  Inputs=|+-
  Sum2 : Sum  Inputs=|--
  Sum3 : Sum  Inputs=|++
  Switch : Switch  Criteria=u2 > Threshold  Threshold=dcVoltage.reqDCBusVoltage*0.8  SaturateOnIntegerOverflow=off  InputSameDT=off
  Voltage control : Subsystem
  Mod : Outport
  wires:
  Voltage control/1(u) -> Sum2/1
  Voref/1 -> Switch/2, Switch/1, Sum/1
  Switch/1 -> Divide/2
  Sum2/1 -> Current control/1(e)
  Vo/1 -> Sum/2
  Current control/1(u) -> Sum3/1
  IL/1 -> Sum2/2
  Sum/1 -> Voltage control/1(e)
  Sum3/1 -> Saturation/1
  Saturation/1 -> Mod/1
  Constant/1 -> Switch/3
  Divide/1 -> Sum3/2
  Vbat/1 -> Divide/1

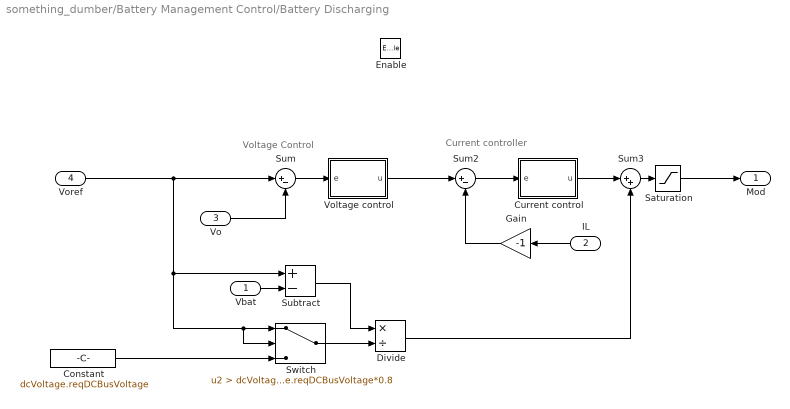
== system something_dumber/Battery Management Control/Battery Discharging ==
  note: Current controller
  note: Voltage Control
  Vbat : Inport
  IL : Inport  Port=2
  Vo : Inport  Port=3
  Voref : Inport  Port=4
  Enable : EnablePort  StatesWhenEnabling=reset
  Constant : Constant  Value=dcVoltage.reqDCBusVoltage
  Current control : Subsystem
  Divide : Product  Inputs=*/
  Gain : Gain  Gain=-1
  Saturation : Saturate  UpperLimit=1  LowerLimit=0
  Subtract : Sum  Inputs=+-
  Sum : Sum  Inputs=|+-
  Sum2 : Sum  Inputs=|+-
  Sum3 : Sum  Inputs=|++
  Switch : Switch  Criteria=u2 > Threshold  Threshold=dcVoltage.reqDCBusVoltage*0.8  SaturateOnIntegerOverflow=off  InputSameDT=off
  Voltage control : Subsystem
  Mod : Outport
  wires:
  Voltage control/1(u) -> Sum2/1
  Voref/1 -> Sum/1, Subtract/1, Switch/2, Switch/1
  Switch/1 -> Divide/2
  Subtract/1 -> Divide/1
  Sum2/1 -> Current control/1(e)
  Vo/1 -> Sum/2
  Current control/1(u) -> Sum3/1
  IL/1 -> Gain/1
  Sum/1 -> Voltage control/1(e)
  Sum3/1 -> Saturation/1
  Saturation/1 -> Mod/1
  Vbat/1 -> Subtract/2
  Constant/1 -> Switch/3
  Gain/1 -> Sum2/2
  Divide/1 -> Sum3/2

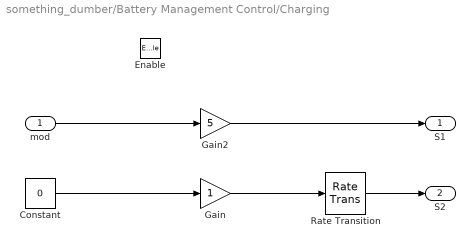
== system something_dumber/Battery Management Control/Charging ==
  mod : Inport
  Enable : EnablePort  StatesWhenEnabling=reset
  Constant : Constant  Value=0
  Gain : Gain
  Gain2 : Gain  Gain=5
  Rate Transition : RateTransition
  S1 : Outport
  S2 : Outport  Port=2
  wires:
  mod/1 -> Gain2/1
  Gain2/1 -> S1/1
  Constant/1 -> Gain/1
  Gain/1 -> Rate Transition/1
  Rate Transition/1 -> S2/1

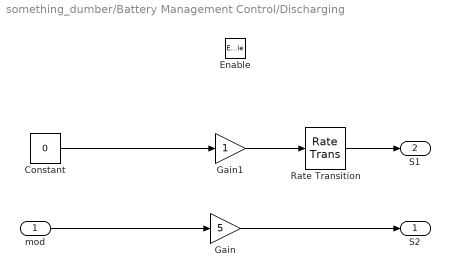
== system something_dumber/Battery Management Control/Discharging ==
  mod : Inport
  Enable : EnablePort  StatesWhenEnabling=reset
  Constant : Constant  Value=0
  Gain : Gain  Gain=5
  Gain1 : Gain
  Rate Transition : RateTransition
  S2 : Outport
  S1 : Outport  Port=2
  wires:
  mod/1 -> Gain/1
  Gain/1 -> S2/1
  Constant/1 -> Gain1/1
  Gain1/1 -> Rate Transition/1
  Rate Transition/1 -> S1/1

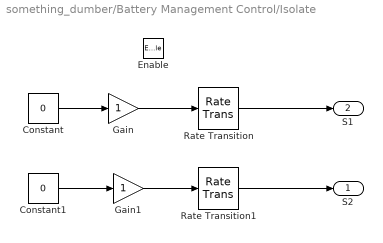
== system something_dumber/Battery Management Control/Isolate ==
  Enable : EnablePort  StatesWhenEnabling=reset
  Constant : Constant  Value=0
  Constant1 : Constant  Value=0
  Gain : Gain
  Gain1 : Gain
  Rate Transition : RateTransition
  Rate Transition1 : RateTransition
  S2 : Outport
  S1 : Outport  Port=2
  wires:
  Constant/1 -> Gain/1
  Constant1/1 -> Gain1/1
  Gain/1 -> Rate Transition/1
  Gain1/1 -> Rate Transition1/1
  Rate Transition/1 -> S1/1
  Rate Transition1/1 -> S2/1

== system something_dumber/Battery Management Control/PWM ==
  mod : Inport
  PWM Generator : eePwmGenerator/PWM Generator  CarrCount=Up  Tper=1/bms.batteryConverterSwitchingFrequency  Tdelay=0  Ts=1/(10*bms.batteryConverterSwitchingFrequency)
  Rate Transition1 : RateTransition  OutPortSampleTime=1/(10*bms.batteryConverterSwitchingFrequency)
  PWM : Outport
  wires:
  Rate Transition1/1 -> PWM Generator/1
  mod/1 -> Rate Transition1/1
  PWM Generator/1 -> PWM/1

== system something_dumber/Load/AC Current Sensor2 ==
  Current Sensor : fl_lib/Electrical/Electrical Sensors/Current Sensor
  PS-Simulink Converter : nesl_utility/PS-Simulink Converter  PhysicalDomain=network_engine_domain  SubClassName=ps_output  LeftPortType=input  RightPortType=output  PseudoPeriodic=off  Frequencies=[]  VectorFormat=1-D array  Unit=1  AffineConversion=off
  Scope : Scope
      settings: ActiveDisplayYMinimum=-2.69141  ActiveDisplayYMaximum=24.19807  DataLoggingVariableName=ScopeData4
  Sensor dynamics : TransferFcn  Numerator=1  Denominator=[1/sensor.samplingFreq 1]
  - : PMIOPort  Side=Left
  + : PMIOPort  Port=2  Side=Right
  tag scope: Iload=global
  wires:
  PS-Simulink Converter/1 -> Sensor dynamics/1
  Sensor dynamics/1 -> Scope/1, [Iload]
  connections:
  Current Sensor/RConn1 -- PS-Simulink Converter/LConn1
  +/RConn1 -- Current Sensor/LConn1
  Current Sensor/RConn2 -- -/RConn1

== system something_dumber/Load/Load ==
  " " : Constant
  " 1" : Constant  Value=1.5
  " 2" : Constant  Value=dcVoltage.reqDCBusVoltage*dcVoltage.reqDCBusVoltage*1e-3
  Divide : Product  Inputs=*/
  Load Power (kW) : Gain  Gain=lunarCase.P_kW
  Simulink-PS Converter1 : nesl_utility/Simulink-PS Converter  PhysicalDomain=network_engine_domain  SubClassName=ps_input  LeftPortType=input  RightPortType=output  PseudoPeriodic=off  Frequencies=[]  NoiseDistribution=none  NoiseParameters=[]  Unit=1  AffineConversion=off  FilteringAndDerivatives=provide  SimscapeFilterOrder=1  InputFilterTimeConstant=0.001  UdotUserProvided=0
  Switch : Switch  Criteria=u2 > Threshold  SaturateOnIntegerOverflow=off  InputSameDT=off
  R : PMIOPort  Side=Right
  wires:
  " "/1 -> Load Power (kW)/1
  Load Power (kW)/1 -> Switch/1, Switch/2
  " 1"/1 -> Switch/3
  " 2"/1 -> Divide/1
  Switch/1 -> Divide/2
  Divide/1 -> Simulink-PS Converter1/1
  connections:
  Simulink-PS Converter1/RConn1 -- R/RConn1

== system something_dumber/Load/Load Flag ==
  Data Type Conversion1 : DataTypeConversion  SaturateOnIntegerOverflow=off  RndMeth=Floor
  NOT : Logic  Operator=NOT  IconShape=distinctive  AllPortsSameDT=off  OutDataTypeStr=boolean
  OR : Logic  Operator=OR  IconShape=distinctive  AllPortsSameDT=off  OutDataTypeStr=boolean
  Simulink-PS Converter2 : nesl_utility/Simulink-PS Converter  PhysicalDomain=network_engine_domain  SubClassName=ps_input  LeftPortType=input  RightPortType=output  PseudoPeriodic=off  Frequencies=[]  NoiseDistribution=none  NoiseParameters=[]  Unit=1  AffineConversion=off  FilteringAndDerivatives=provide  SimscapeFilterOrder=1  InputFilterTimeConstant=0.001  UdotUserProvided=0
  CB : PMIOPort  Side=Right
  wires:
  [loadShutDown] -> OR/1
  Data Type Conversion1/1 -> Simulink-PS Converter2/1
  [ShutDown] -> OR/2  "System Status"
  OR/1 -> NOT/1
  NOT/1 -> Data Type Conversion1/1
  connections:
  Simulink-PS Converter2/RConn1 -- CB/RConn1

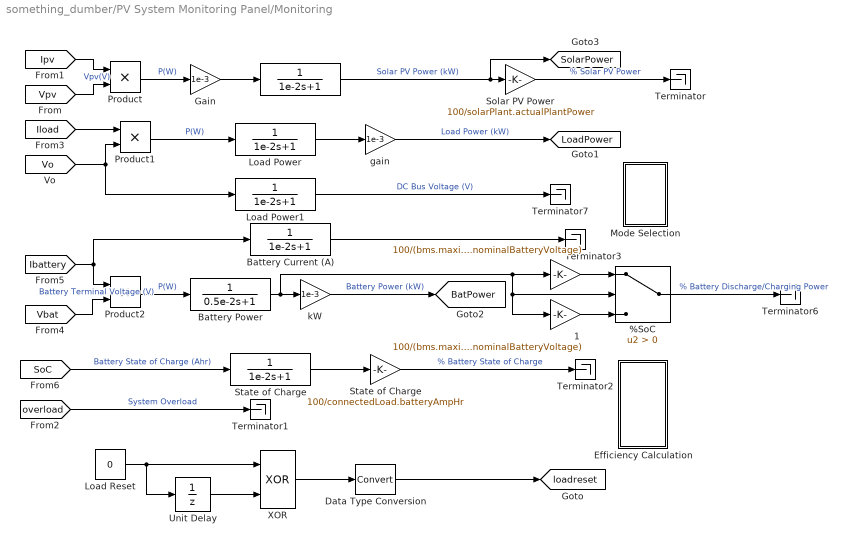
== system something_dumber/PV System Monitoring Panel/Monitoring ==
  " " : Gain  Gain=100/(bms.maximumChargingCurrentLimit*battery.nominalBatteryVoltage)
  "  " : TransferFcn  Denominator=[1e-2 1]
  " 1" : Gain  Gain=100/(bms.maximumDisChargingCurrent*battery.nominalBatteryVoltage)
  " State of Charge" : Gain  Gain=100/connectedLoad.batteryAmpHr
  %SoC : Switch  Criteria=u2 > Threshold  SaturateOnIntegerOverflow=off  InputSameDT=off
  Battery Current (A) : TransferFcn  Denominator=[1e-2 1]
  Battery Power : TransferFcn  Denominator=[0.5e-2 1]
  Data Type Conversion : DataTypeConversion  SaturateOnIntegerOverflow=off  RndMeth=Floor
  Efficiency Calculation : Subsystem
  Gain : Gain  Gain=1e-3
  Load Power : TransferFcn  Denominator=[1e-2 1]
  Load Power1 : TransferFcn  Denominator=[1e-2 1]
  Load Reset : Constant  Value=0
  Mode Selection : Subsystem
  Product : Product
  Product1 : Product
  Product2 : Product
  Solar PV Power : Gain  Gain=100/solarPlant.actualPlantPower
  State of Charge : TransferFcn  Denominator=[1e-2 1]
  Terminator{,1..3,6..7} (6 alike) : Terminator
  Unit Delay : UnitDelay  SampleTime=1e-3
  XOR : Logic  Operator=XOR  IconShape=distinctive  AllPortsSameDT=off  OutDataTypeStr=boolean
  gain : Gain  Gain=1e-3
  kW : Gain  Gain=1e-3
  tag scope: BatPower=global, LoadPower=global, SolarPower=global, loadreset=global
  wires:
  [Vpv] -> Product/2  "Vpv(V)"
  Load Power/1 -> gain/1
  Product1/1 -> Load Power/1  "P(W)"
  [Vbat] -> Product2/2  "Battery Terminal Voltage (V)"
  [Iload] -> Product1/1
  Battery Power/1 -> kW/1, " 1"/1, %SoC/2, " "/1
  "  "/1 -> [SolarPower], Solar PV Power/1  "Solar PV Power (kW)"
  [Ibattery] -> Product2/1, Battery Current (A)/1
  Product2/1 -> Battery Power/1  "P(W)"
  [Ipv] -> Product/1
  [Vo] -> Product1/2, Load Power1/1
  Product/1 -> Gain/1  "P(W)"
  [SoC] -> State of Charge/1  "Battery State of Charge (Ahr)"
  Solar PV Power/1 -> Terminator/1  "% Solar PV Power"
  gain/1 -> [LoadPower]  "Load Power (kW)"
  kW/1 -> [BatPower]  "Battery Power (kW)"
  State of Charge/1 -> " State of Charge"/1
  " State of Charge"/1 -> Terminator2/1  "% Battery State of Charge"
  " "/1 -> %SoC/1
  " 1"/1 -> %SoC/3
  %SoC/1 -> Terminator6/1  "% Battery Discharge/Charging Power"
  Battery Current (A)/1 -> Terminator3/1
  Gain/1 -> "  "/1
  Load Power1/1 -> Terminator7/1  "DC Bus Voltage (V)"
  [overload] -> Terminator1/1  "System Overload"
  XOR/1 -> Data Type Conversion/1
  Load Reset/1 -> XOR/1, Unit Delay/1
  Unit Delay/1 -> XOR/2
  Data Type Conversion/1 -> [loadreset]

== system something_dumber/Battery Management Control/Battery Charging/Current control ==
  e : Inport
  1/T : Gain  Gain=1/bms.chargeCurrentZeroTimeConst
  Integrator : Integrator  LimitOutput=on  UpperSaturationLimit=1.3  LowerSaturationLimit=-1.3
  Kp : Gain  Gain=bms.chargeCurrentGain
  Saturation : Saturate  UpperLimit=1.5  LowerLimit=-1.5
  Sum7 : Sum  Inputs=|++
  u : Outport  VectorParamsAs1DForOutWhenUnconnected=off
  wires:
  Integrator/1 -> Sum7/2
  Saturation/1 -> u/1
  Sum7/1 -> Saturation/1
  e/1 -> Kp/1
  Kp/1 -> 1/T/1, Sum7/1
  1/T/1 -> Integrator/1

== system something_dumber/Battery Management Control/Battery Charging/Voltage control ==
  e : Inport
  1/T : Gain  Gain=1/bmsController.chosenChargeVoltageZeroTimeConst
  Integrator : Integrator  LimitOutput=on  UpperSaturationLimit=bms.maximumChargingCurrentLimit  LowerSaturationLimit=-1*bms.maximumChargingCurrentLimit
  Kp : Gain  Gain=bmsController.chosenChargeVoltageGain
  Saturation : Saturate  UpperLimit=bms.maximumChargingCurrentLimit  LowerLimit=-1*bms.maximumChargingCurrentLimit
  Sum7 : Sum  Inputs=|++
  u : Outport  VectorParamsAs1DForOutWhenUnconnected=off
  wires:
  Integrator/1 -> Sum7/2
  Saturation/1 -> u/1
  e/1 -> Kp/1
  Kp/1 -> 1/T/1, Sum7/1
  1/T/1 -> Integrator/1
  Sum7/1 -> Saturation/1

== system something_dumber/Battery Management Control/Battery Discharging/Current control ==
  e : Inport
  1/T : Gain  Gain=1/bms.dischargeCurrentZeroTimeConst
  Integrator : Integrator  InitialCondition=1  LimitOutput=on  UpperSaturationLimit=1  LowerSaturationLimit=-0.5
  Kp : Gain  Gain=bms.dischargeCurrentGain
  Saturation : Saturate  UpperLimit=1  LowerLimit=-1
  Sum7 : Sum  Inputs=|++
  u : Outport  VectorParamsAs1DForOutWhenUnconnected=off
  wires:
  Integrator/1 -> Sum7/2
  Saturation/1 -> u/1
  Sum7/1 -> Saturation/1
  e/1 -> Kp/1
  Kp/1 -> 1/T/1, Sum7/1
  1/T/1 -> Integrator/1

== system something_dumber/Battery Management Control/Battery Discharging/Voltage control ==
  e : Inport
  1/T : Gain  Gain=1/bmsController.chosenDischargeVoltageZeroTimeConst
  Integrator : Integrator  LimitOutput=on  UpperSaturationLimit=bms.maximumDisChargingCurrent  LowerSaturationLimit=-1*bms.maximumDisChargingCurrent
  Kp : Gain  Gain=bmsController.chosenDischargeVoltageGain
  Saturation : Saturate  UpperLimit=bms.maximumDisChargingCurrent  LowerLimit=-1*bms.maximumDisChargingCurrent
  Sum7 : Sum  Inputs=|++
  u : Outport  VectorParamsAs1DForOutWhenUnconnected=off
  wires:
  Integrator/1 -> Sum7/2
  Saturation/1 -> u/1
  e/1 -> Kp/1
  Kp/1 -> 1/T/1, Sum7/1
  1/T/1 -> Integrator/1
  Sum7/1 -> Saturation/1

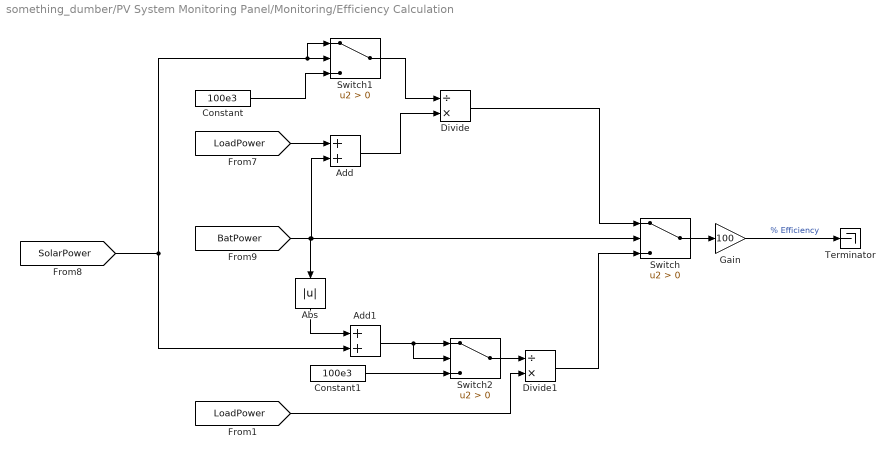
== system something_dumber/PV System Monitoring Panel/Monitoring/Efficiency Calculation ==
  Abs : Abs  SaturateOnIntegerOverflow=off
  Add : Sum
  Add1 : Sum
  Constant : Constant  Value=100e3
  Constant1 : Constant  Value=100e3
  Divide : Product  Inputs=/*
  Divide1 : Product  Inputs=/*
  Gain : Gain  Gain=100
  Switch : Switch  Criteria=u2 > Threshold  SaturateOnIntegerOverflow=off  InputSameDT=off
  Switch1 : Switch  Criteria=u2 > Threshold  SaturateOnIntegerOverflow=off  InputSameDT=off
  Switch2 : Switch  Criteria=u2 > Threshold  SaturateOnIntegerOverflow=off  InputSameDT=off
  Terminator : Terminator
  wires:
  [BatPower] -> Abs/1, Add/2, Switch/2
  [LoadPower] -> Add/1
  [SolarPower] -> Switch1/1, Switch1/2, Add1/2
  Constant/1 -> Switch1/3
  Switch1/1 -> Divide/1
  Add/1 -> Divide/2
  Abs/1 -> Add1/1
  [LoadPower] -> Divide1/2
  Add1/1 -> Switch2/2, Switch2/1
  Constant1/1 -> Switch2/3
  Switch2/1 -> Divide1/1
  Divide/1 -> Switch/1
  Divide1/1 -> Switch/3
  Switch/1 -> Gain/1
  Gain/1 -> Terminator/1  "% Efficiency"

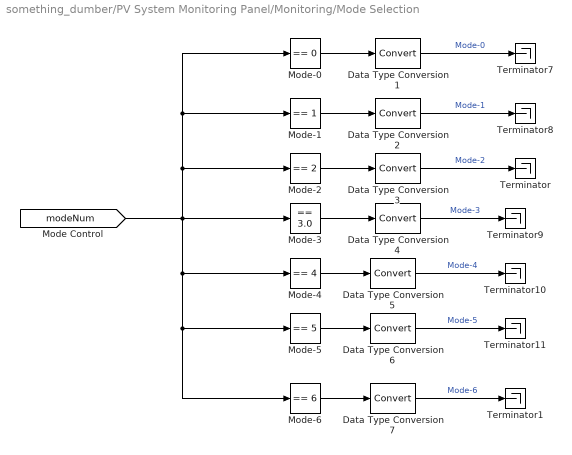
== system something_dumber/PV System Monitoring Panel/Monitoring/Mode Selection ==
  Data Type Conversion{1..7} (7 alike) : DataTypeConversion  SaturateOnIntegerOverflow=off  RndMeth=Floor
  Mode-0 : simulink/Logic and Bit Operations/Compare To Constant  relop===  const=0  OutDataTypeStr=boolean
  Mode-1 : simulink/Logic and Bit Operations/Compare To Constant  relop===  const=1  OutDataTypeStr=boolean
  Mode-2 : simulink/Logic and Bit Operations/Compare To Constant  relop===  const=2  OutDataTypeStr=boolean
  Mode-3 : simulink/Logic and Bit Operations/Compare To Constant  relop===  const=3.0  OutDataTypeStr=boolean
  Mode-4 : simulink/Logic and Bit Operations/Compare To Constant  relop===  const=4  OutDataTypeStr=boolean
  Mode-5 : simulink/Logic and Bit Operations/Compare To Constant  relop===  const=5  OutDataTypeStr=boolean
  Mode-6 : simulink/Logic and Bit Operations/Compare To Constant  relop===  const=6  OutDataTypeStr=boolean
  Terminator{,1,7..11} (7 alike) : Terminator
  wires:
  Mode-0/1 -> Data Type Conversion1/1
  Mode-3/1 -> Data Type Conversion4/1
  [modeNum] -> Mode-3/1, Mode-4/1, Mode-5/1, Mode-6/1, Mode-2/1, Mode-1/1, Mode-0/1
  Mode-4/1 -> Data Type Conversion5/1
  Mode-1/1 -> Data Type Conversion2/1
  Mode-2/1 -> Data Type Conversion3/1
  Mode-5/1 -> Data Type Conversion6/1
  Mode-6/1 -> Data Type Conversion7/1
  Data Type Conversion1/1 -> Terminator7/1  "Mode-0"
  Data Type Conversion2/1 -> Terminator8/1  "Mode-1"
  Data Type Conversion3/1 -> Terminator/1  "Mode-2"
  Data Type Conversion4/1 -> Terminator9/1  "Mode-3"
  Data Type Conversion5/1 -> Terminator10/1  "Mode-4"
  Data Type Conversion6/1 -> Terminator11/1  "Mode-5"
  Data Type Conversion7/1 -> Terminator1/1  "Mode-6"

== matlab function something_dumber/PV_MPPT_6module ==
  settings: updateMethod=DISCRETE
  data: G input; Ibus output; T input; Vbus input; en input; VmpT input; ImpT input; Pbus output; Pavail output; Vpv output; Ipv output; Imod output; duty output
function [Ibus, Pbus, Pavail, Vpv, Ipv, Imod, duty] = fcn(G,T,Vbus,en,VmpT,ImpT)
%#codegen
% EOL teammate MPP data; illustrative piecewise I-V fit.
% Shared PV bus, single coordinated P&O, six averaged PI branches.
persistent Vcmd dir Pprev count il integ
if isempty(Vcmd)
 Vcmd=217; dir=1; Pprev=0; count=0; il=zeros(6,1); integ=zeros(6,1);
end
dt=1e-4; eta=0.96; Gref=1367;
gs=max(0,min(1.5,G/Gref));
vmp=max(10,VmpT); imp=max(0,ImpT)*gs;
% Curve passes through Isc, Imp at Vmp, and zero at Voc.
% Isc=1.04 Imp, Voc=1.13 Vmp are MODEL ASSUMPTIONS.
isc=1.04*imp; voc=1.13*vmp;
Vcmd=max(0.5*vmp,min(0.99*voc,Vcmd));
if Vcmd<=vmp
 ipv=max(0,isc-(isc-imp)*(Vcmd/vmp)^2);
else
 ipv=max(0,imp*(voc-Vcmd)/(voc-vmp));
end
Ppv=Vcmd*ipv; Pavail=max(0,vmp*imp*eta);
count=count+1;
if count>=100
 if Ppv<Pprev, dir=-dir; end
 Vcmd=Vcmd+dir*0.5; Pprev=Ppv; count=0;
end
% Power-to-current reference; current limited by PV production.
v=max(30,Vbus);
Ptarget=max(0,min(Ppv*eta,Pavail))*max(0,min(1,en));
Iref=Ptarget/v/6;
Imod=zeros(6,1); duty=zeros(6,1);
for k=1:6
 % Averaged current PI with feedforward; shared-array duty proxy.
 err=Iref-il(k);
 dff=Vbus/max(1,1.15*Vcmd);
 d=max(0,min(0.85,dff+0.0015*err+integ(k)));
 % Average inductor dynamics; 33 uH each.
 next=il(k)+dt*(1.15*Vcmd*d-Vbus)/33e-6;
 % Avoid nonphysical reverse PV current.
 next=max(0,next);
 % Anti-windup: integrate only when unsaturated or correcting.
 if (d>0 && d<0.85) || (d<=0 && err>0) || (d>=0.85 && err<0)
  integ(k)=integ(k)+3*dt*err;
 end
 il(k)=next; Imod(k)=next; duty(k)=d;
end
% Conservation clamp: do not inject more power than PV can supply.
Iraw=sum(Imod); Ibus=min(Iraw,Ptarget/v);
Pbus=Ibus*max(0,Vbus); Vpv=Vcmd; Ipv=ipv;
end
